simulink library "DQFeedforward"  (R2026a)
settings: Solver=VariableStepAuto
undefined symbols (not defined in the file): feedforwardCfg, pmsmCfg
settings Model: Creator=24322  LastModifiedBy=24322

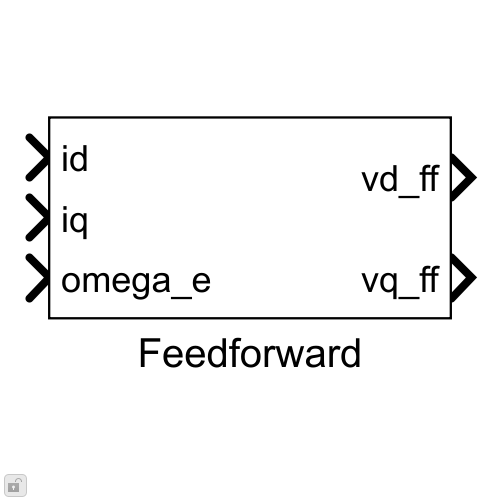
[thumbnail: Simulink's stored preview of the top-level diagram]
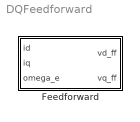
== system DQFeedforward ==
  Feedforward : Subsystem

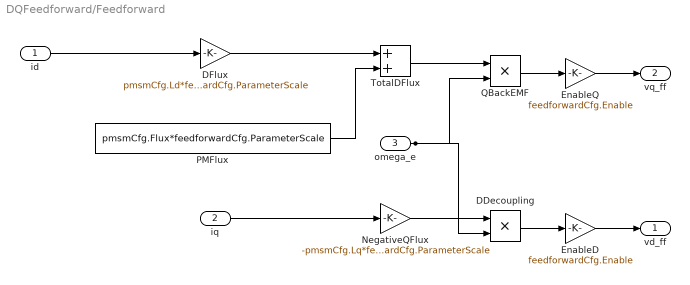
== system DQFeedforward/Feedforward ==
  id : Inport
  iq : Inport  Port=2
  omega_e : Inport  Port=3
  DDecoupling : Product
  DFlux : Gain  Gain=pmsmCfg.Ld*feedforwardCfg.ParameterScale
  EnableD : Gain  Gain=feedforwardCfg.Enable
  EnableQ : Gain  Gain=feedforwardCfg.Enable
  NegativeQFlux : Gain  Gain=-pmsmCfg.Lq*feedforwardCfg.ParameterScale
  PMFlux : Constant  Value=pmsmCfg.Flux*feedforwardCfg.ParameterScale
  QBackEMF : Product
  TotalDFlux : Sum
  vd_ff : Outport
  vq_ff : Outport  Port=2
  wires:
  EnableQ/1 -> vq_ff/1
  EnableD/1 -> vd_ff/1
  QBackEMF/1 -> EnableQ/1
  DDecoupling/1 -> EnableD/1
  TotalDFlux/1 -> QBackEMF/1
  omega_e/1 -> DDecoupling/2, QBackEMF/2
  NegativeQFlux/1 -> DDecoupling/1
  PMFlux/1 -> TotalDFlux/2
  DFlux/1 -> TotalDFlux/1
  id/1 -> DFlux/1
  iq/1 -> NegativeQFlux/1
